simulink model "aerodynamic_model_V1_1_Coupling"  (R2025b)
settings: Solver=ode4  StartTime=0.0  StopTime=8  FixedStep=Ts  RelTol=1e-3
InitFcn:
  | % Run initial_main.m first to load Ad,As,Tq_prop,Tq_mass,...
values from neighbouring files (symbols this model uses):
  alpha_du0_v_tail_L = trim_aero_ic.v_tail_L.alpha_du0    [initial_main_V1_1.m]
  alpha_du0_v_tail_R = trim_aero_ic.v_tail_R.alpha_du0    [initial_main_V1_1.m]
  alpha_du0_wing_L = trim_aero_ic.wing_L.alpha_du0    [initial_main_V1_1.m]
  alpha_du0_wing_R = trim_aero_ic.wing_R.alpha_du0    [initial_main_V1_1.m]
  As = sys_sd.A    [initial_main_V1_1.m]
  BladePitch_deg = 34    [initial_main_V1_1.m]
  Bs = sys_sd.B    [initial_main_V1_1.m]
  Cs = sys_sd.C    [initial_main_V1_1.m]
  ctrl_delta_lim_deg = strips.delta_lim_deg    [initial_main_V1_1.m]
  ctrl_map_aileron_L = aero.wing_L.map_aileron(:)    [initial_main_V1_1.m]
  ctrl_map_aileron_R = aero.wing_R.map_aileron(:)    [initial_main_V1_1.m]
  ctrl_map_tail_L = aero.v_tail_L.map_tail(:)    [initial_main_V1_1.m]
  ctrl_map_tail_R = aero.v_tail_R.map_tail(:)    [initial_main_V1_1.m]
  Ds = sys_sd.D    [initial_main_V1_1.m]
  I_cg_b = R_sb * I_cg_m * R_sb.'    [aeroelastic.m]    (also in initial_main_V1_1.m = grav.I_cg_b)
  I_cg_b_inv = R_sb * I_cg_m_inv * R_sb.'    [aeroelastic.m]    (also in initial_main_V1_1.m = grav.I_cg_b_inv)
  m_total_kg = grav.m_total_kg    [initial_main_V1_1.m]
  n_modes = size(Phi, 2)    [aeroelastic.m]    (also in initial_main_V1_1.m = n_rigid + n_elastic)
  ones_1_tail = ones(1, size(r_cg2ac_b_v_tail_L, 2))    [initial_main_V1_1.m]
  ones_1_wing = ones(1, size(r_cg2ac_b_wing_L, 2))    [initial_main_V1_1.m]
  polar_alpha_deg = polar.alpha_deg(:).'    [initial_main_V1_1.m]
  polar_CD = polar.CD(:).'    [initial_main_V1_1.m]
  polar_CDp = polar.CDp(:).'    [initial_main_V1_1.m]
  polar_CL = polar.CL(:).'    [initial_main_V1_1.m]
  polar_CM = polar.CM(:).'    [initial_main_V1_1.m]
  r_cg2ac_b_v_tail_L = R_sb * aero.v_tail_L.r_ac_s    [initial_main_V1_1.m]
  r_cg2ac_b_v_tail_R = R_sb * aero.v_tail_R.r_ac_s    [initial_main_V1_1.m]
  r_cg2ac_b_wing_L = R_sb * aero.wing_L.r_ac_s    [initial_main_V1_1.m]
  r_cg2ac_b_wing_R = R_sb * aero.wing_R.r_ac_s    [initial_main_V1_1.m]
  r_cg2kink_b = eng.r_cg2kink_b    [initial_main_V1_1.m]
  r_cg2node_b = aeroelastic.node_arms(nodes, 'R_sb', R_sb).r_cg2node_b    [initial_main_V1_1.m]
  T_aero2W = aeroelastic.wing_aileron_to_W(strips).T    [initial_main_V1_1.m]
  T_prop2W = load_maps.T_prop2W    [initial_main_V1_1.m]
  Tq_mass = load_maps.Tq_mass    [initial_main_V1_1.m]
  trim_Attitude_rad0 = trim_default.Attitude_rad0    [initial_main_V1_1.m]
  trim_Omega_b0 = trim_default.Omega_b0    [initial_main_V1_1.m]
  trim_Position0 = trim_default.Position0    [initial_main_V1_1.m]
  trim_Velocity_b0 = trim_default.Velocity_b0    [initial_main_V1_1.m]
  Ts = 0.001    [initial_main_V1_1.m]
  U = 50    [initial_main_V1_1.m]
  v_tail_cant_rad = deg2rad(v_tail_cant_deg)    [initial_main_V1_1.m]
  W_mass_g = grav.W_mass    [initial_main_V1_1.m]
  x0_structure = trim_default.x0_structure    [initial_main_V1_1.m]
  x0_wagner_v_tail_L = trim_aero_ic.v_tail_L.x0_wagner    [initial_main_V1_1.m]
  x0_wagner_v_tail_R = trim_aero_ic.v_tail_R.x0_wagner    [initial_main_V1_1.m]
  x0_wagner_wing_L = trim_aero_ic.wing_L.x0_wagner    [initial_main_V1_1.m]
  x0_wagner_wing_R = trim_aero_ic.wing_R.x0_wagner    [initial_main_V1_1.m]
undefined symbols (not defined in the file or in its folder): Ad_v_tail_L, Ad_v_tail_R, Ad_wing_L, Ad_wing_R, Bd_v_tail_L, Bd_v_tail_R, Bd_wing_L, Bd_wing_R, c_over_2U_v_tail_L, c_over_2U_v_tail_R, c_over_2U_wing_L, c_over_2U_wing_R, Cd_v_tail_L, Cd_v_tail_R, Cd_wing_L, Cd_wing_R, Dd_v_tail_L, Dd_v_tail_R, Dd_wing_L, Dd_wing_R, G_du_v_tail_L, G_du_v_tail_R, G_du_wing_L, G_du_wing_R, polar_aileron_alpha_deg, polar_aileron_dCD, polar_aileron_dCL, polar_aileron_dCM, polar_aileron_delta_deg, polar_ruddervator_alpha_deg, polar_ruddervator_dCD, polar_ruddervator_dCL, polar_ruddervator_dCM, polar_ruddervator_delta_deg, qS_strip_v_tail_L, qS_strip_v_tail_R, qS_strip_wing_L, qS_strip_wing_R, qSc_strip_v_tail_L, qSc_strip_v_tail_R, qSc_strip_wing_L, qSc_strip_wing_R, T_m2b_v_tail_L, T_m2b_v_tail_R, T_m2b_wing_L, T_m2b_wing_R, T_m2h_v_tail_L, T_m2h_v_tail_R, T_m2h_wing_L, T_m2h_wing_R, Tq_CM_v_tail_L, Tq_CM_v_tail_R, Tq_CM_wing_L, Tq_CM_wing_R, Tq_D_v_tail_L, Tq_D_v_tail_R, Tq_D_wing_L, Tq_D_wing_R, Tq_v_tail_L, Tq_v_tail_R ... (+2)
libraries: Prop_gryo x9, matrix_library x2
(part 1 of 2)
settings Model: Creator=someone  LastModifiedBy=someone
settings DataIOCC: ExternalInput=trim_input_dataset  LoadExternalInput=on

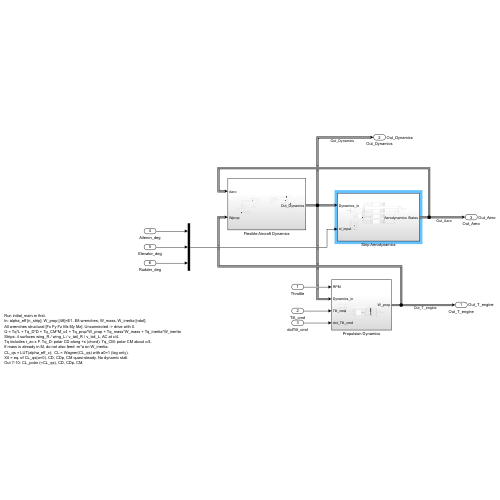
[thumbnail: Simulink's stored preview of the top-level diagram]
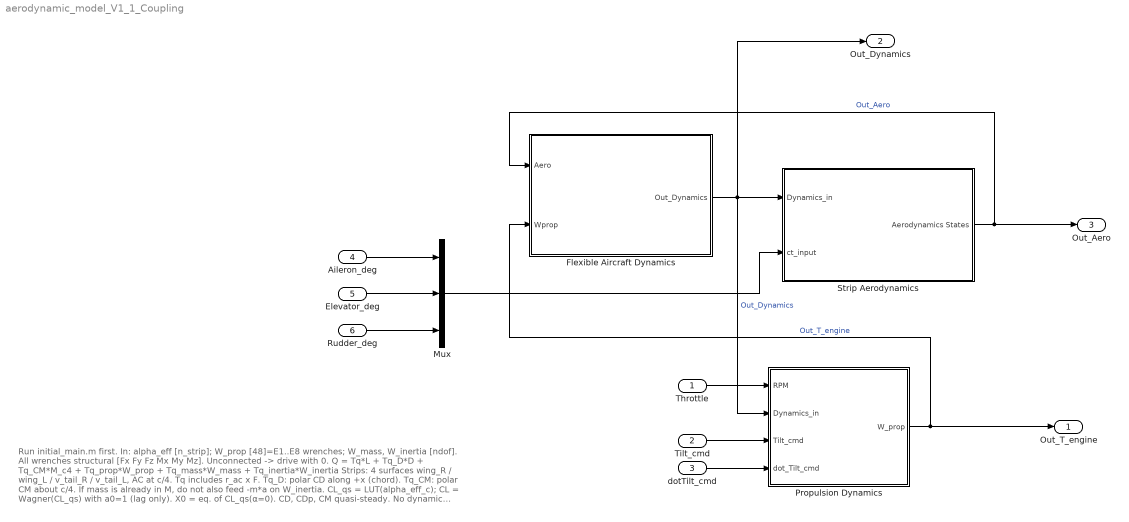
== system aerodynamic_model_V1_1_Coupling ==
  note: Run initial_main.m first.
      | In: alpha_eff [n_strip]; W_prop [48]=E1..E8 wrenches; W_mass, W_inertia [ndof].
      | All wrenches structural [Fx Fy Fz Mx My Mz]. Unconnected -> drive with 0.
      | Q = Tq*L + Tq_D*D + Tq_CM*M_c4 + Tq_prop*W_prop + Tq_mass*W_mass + Tq_inertia*W_inertia
      | Strips: 4 surfaces wing_R / wing_L / v_tail_R / v_tail_L, AC at c/4.
      | Tq includes r_ac x F. Tq_D: polar CD along +x (chord). Tq_CM: polar CM about c/4.
      | If mass is already in M, do not also feed -m*a on W_inertia.
      | CL_qs = LUT(alpha_eff_c);  CL = Wagner(CL_qs) with a0=1 (lag only).
      | X0 = eq. of CL_qs(α=0). CD, CDp, CM quasi-steady. No dynamic stall.
      | Out 7-10: CL_polar (=CL_qs), CD, CDp, CM.
  Throttle : Inport  PortDimensions=8
  Tilt_cmd : Inport  Port=2  PortDimensions=8
  dotTilt_cmd : Inport  Port=3  PortDimensions=8
  Aileron_deg : Inport  Port=4
  Elevator_deg : Inport  Port=5
  Rudder_deg : Inport  Port=6
  Flexible Aircraft Dynamics : Subsystem
  Mux : Mux  Inputs=3
  Propulsion Dynamics : Subsystem
  Strip Aerodynamics : Subsystem
  Out_T_engine : Outport  SignalName=Out_T_engine
  Out_Dynamics : Outport  Port=2  SignalName=Out_Dynamics
  Out_Aero : Outport  Port=3  SignalName=Out_Aero
  wires:
  Throttle/1 -> Propulsion Dynamics/1(RPM)
  Tilt_cmd/1 -> Propulsion Dynamics/3(Tilt_cmd)
  dotTilt_cmd/1 -> Propulsion Dynamics/4(dot_Tilt_cmd)
  Flexible Aircraft Dynamics/1(Out_Dynamics) -> Out_Dynamics/1, Strip Aerodynamics/1(Dynamics_in), Propulsion Dynamics/2(Dynamics_in)  "Out_Dynamics"
  Strip Aerodynamics/1(Aerodynamics States) -> Out_Aero/1, Flexible Aircraft Dynamics/1(Aero)  "Out_Aero"
  Propulsion Dynamics/1(W_prop) -> Out_T_engine/1, Flexible Aircraft Dynamics/2(Wprop)  "Out_T_engine"
  Aileron_deg/1 -> Mux/1
  Rudder_deg/1 -> Mux/3
  Mux/1 -> Strip Aerodynamics/2(ct_input)
  Elevator_deg/1 -> Mux/2

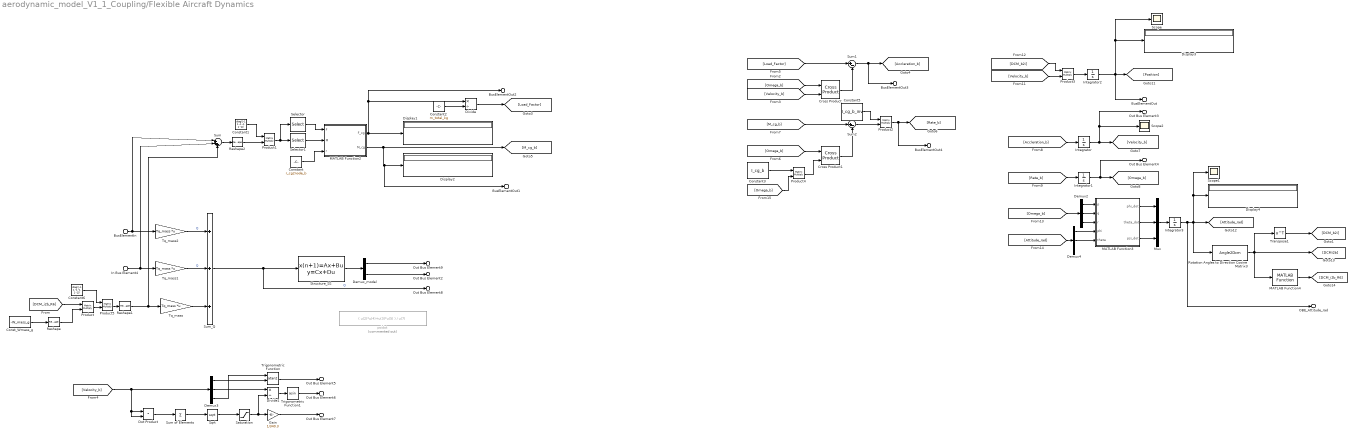
== system aerodynamic_model_V1_1_Coupling/Flexible Aircraft Dynamics ==
  BusElementIn : Inport  PortName=Aero  Element=W_aero_S
  In Bus Element4 : Inport  Port=2  PortName=Wprop  Element=W_m
  Const_Wmass_g : Constant  Value=-W_mass_g
  Constant : Constant  Value=r_cg2node_b
  Constant1 : Constant  Value=diag([-1 1 -1 -1 1 -1])
  Constant2 : Constant  Value=m_total_kg
  Constant3 : Constant  Value=I_cg_b
  Constant5 : Constant  Value=I_cg_b_inv
  Constant6 : Constant  Value=diag([-1 1 -1 -1 1 -1])
  Cross Product : matrix_library/Cross Product
  Cross Product1 : matrix_library/Cross Product
  Demux2 : Demux  Outputs=3
  Demux3 : Demux  Outputs=3
  Demux4 : Demux  Outputs=3
  Demux_modal : Demux  Outputs=[n_modes n_modes]
  Display{1..4} (4 alike) : Display
  Divide : Product  Inputs=*/
  Divide1 : Product  Inputs=*/
  Dot Product : DotProduct  OutDataTypeStr=Inherit: Inherit via internal rule
  Gain : Gain  Gain=1/340.3
  Integrator : Integrator  InitialCondition=trim_Velocity_b0
  Integrator1 : Integrator  InitialCondition=trim_Omega_b0
  Integrator2 : Integrator  InitialCondition=trim_Position0
  Integrator3 : Integrator  InitialCondition=trim_Attitude_rad0
  MATLAB Function2 : MATLAB Function  TreatAsAtomicUnit=on
  MATLAB Function3 : MATLAB Function  TreatAsAtomicUnit=on
  MATLAB Function4 : Prop_gryo/Prop1/MATLAB Function  SystemSampleTime=-1  VariantActivationTime=update diagram  EmptyChoice=off  PassThrough=off  PassThroughVariantControl=(default)  EmptyChoiceVariantControl=(default)  AllowFlexibleInterface=on  Latency=0  AutoFrameSizeCalculation=off
  Mux : Mux  Inputs=3
  Product{,1..5} (6 alike) : Product  Multiplication=Matrix(*)
  Reshape : Reshape  OutputDimensionality=Customize  OutputDimensions=[6 89]
  Reshape1 : Reshape
  Reshape2 : Reshape  OutputDimensionality=Customize  OutputDimensions=[6 89]
  Rotation Angles to Direction Cosine Matrix3 : Angle2Dcm
      settings: AttributesFormatString=Rotation Order: %<rotationOrder>
  Saturation : Saturate  UpperLimit=inf  LowerLimit=1e-6
  Scope : Scope
      settings: ActiveDisplayYMinimum=-1  ActiveDisplayYMaximum=1
  Scope1 : Scope
      settings: ActiveDisplayYMinimum=-1  ActiveDisplayYMaximum=1
  Scope2 : Scope
      settings: ActiveDisplayYMinimum=-1  ActiveDisplayYMaximum=1  DataLoggingVariableName=ScopeData2
  Selector : Selector  NumberOfDimensions=2  InputPortWidth=3  IndexOptions=Index vector (dialog),Index vector (dialog)  Indices=[1:3],[1:89]  OutputSizes=1,1
  Selector1 : Selector  NumberOfDimensions=2  InputPortWidth=3  IndexOptions=Index vector (dialog),Index vector (dialog)  Indices=[4:6],[1:89]  OutputSizes=1,1
  Sqrt : Sqrt
  Structure_SS : DiscreteStateSpace  A=As  B=Bs  C=Cs  D=Ds  InitialCondition=x0_structure  SampleTime=Ts
  Sum : Sum  Inputs=|+++
  Sum of Elements : Sum  Inputs=+
  Sum1 : Sum  Inputs=|+-
  Sum2 : Sum  Inputs=|+-
  Sum_Q : Sum  Inputs=+++
  Tq_mass : Gain  Gain=Tq_mass  Multiplication=Matrix(K*u)
  Tq_mass1 : Gain  Gain=Tq_mass  Multiplication=Matrix(K*u)
  Tq_mass2 : Gain  Gain=Tq_mass  Multiplication=Matrix(K*u)
  Transpose1 : Math  Operator=transpose
  Trigonometric Function : Trigonometry  Operator=atan2
  Trigonometric Function1 : Trigonometry  Operator=asin
  psidot : Fcn  Commented=on  Expr=( u(2)*u(4)+u(3)*u(5) ) / u(7)
  Out Bus Element2 : Outport  PortName=Out_Dynamics  Element=elastic_m_velocity
  Out Bus Element3 : Outport  PortName=Out_Dynamics  Element=Velocity_b
  Out Bus Element4 : Outport  PortName=Out_Dynamics  Element=Omega_b
  Out Bus Element5 : Outport  PortName=Out_Dynamics  Element=Alpha
  Out Bus Element6 : Outport  PortName=Out_Dynamics  Element=Beta
  Out Bus Element7 : Outport  PortName=Out_Dynamics  Element=mach
  Out Bus Element8 : Outport  PortName=Out_Dynamics  Element=Q
  Out Bus Element9 : Outport  PortName=Out_Dynamics  Element=elastic_displacement
  OBE_Attitude_rad : Outport  PortName=Out_Dynamics  Element=Attitude_rad
  BusElementOut : Outport  PortName=Out_Dynamics  Element=Position
  BusElementOut1 : Outport  PortName=Out_Dynamics  Element=M_cg
  BusElementOut2 : Outport  PortName=Out_Dynamics  Element=F_cg
  BusElementOut3 : Outport  PortName=Out_Dynamics  Element=Acc_b
  BusElementOut4 : Outport  PortName=Out_Dynamics  Element=Rate_b
  wires:
  Dot Product/1 -> Sum of Elements/1
  [Velocity_b] -> Demux3/1, Dot Product/2, Dot Product/1
  Demux3/3 -> Trigonometric Function/1
  Sum_Q/1 -> Structure_SS/1, Out Bus Element8/1  "Q"
  In Bus Element4/1 -> Tq_mass1/1, Sum/2
  Demux_modal/2 -> Out Bus Element2/1
  Demux_modal/1 -> Out Bus Element9/1
  Tq_mass/1 -> Sum_Q/3
  Sum of Elements/1 -> Sqrt/1
  Demux3/2 -> Divide1/1
  Structure_SS/1 -> Demux_modal/1
  Divide1/1 -> Trigonometric Function1/1
  Demux3/1 -> Trigonometric Function/2
  Const_Wmass_g/1 -> Reshape/1
  Sqrt/1 -> Saturation/1
  Saturation/1 -> Gain/1, Divide1/2
  Trigonometric Function/1 -> Out Bus Element5/1
  Trigonometric Function1/1 -> Out Bus Element6/1
  Gain/1 -> Out Bus Element7/1
  Tq_mass1/1 -> Sum_Q/2  "Q"
  BusElementIn/1 -> Sum/1, Tq_mass2/1
  Tq_mass2/1 -> Sum_Q/1  "Q"
  [DCM_i2b_R6] -> Product/1
  Reshape/1 -> Product/2
  Product5/1 -> Reshape1/1
  Reshape1/1 -> Tq_mass/1, Sum/3
  Sum/1 -> Reshape2/1
  Reshape2/1 -> Product1/2
  Selector/1 -> MATLAB Function2/1(F)
  Selector1/1 -> MATLAB Function2/2(M)
  Constant/1 -> MATLAB Function2/3(r)
  Constant1/1 -> Product1/1
  Product1/1 -> Selector1/1, Selector/1
  MATLAB Function2/1(F_cg) -> Divide/1, BusElementOut2/1, Display1/1
  MATLAB Function2/2(M_cg) -> BusElementOut1/1, Display2/1, [M_cg_b]
  [Omega_b] -> Cross Product/1
  [Velocity_b] -> Cross Product/2
  [Load_Factor] -> Sum1/1
  Cross Product/1 -> Sum1/2
  Constant2/1 -> Divide/2
  Divide/1 -> [Load_Factor]
  Sum1/1 -> BusElementOut3/1, [Accleration_b]
  [Omega_b] -> Cross Product1/1
  Constant3/1 -> Product4/1
  [M_cg_b] -> Sum2/1
  Cross Product1/1 -> Sum2/2
  [Accleration_b] -> Integrator/1
  [Rate_b] -> Integrator1/1
  Integrator/1 -> Scope2/1, Out Bus Element3/1, [Velocity_b]
  Integrator1/1 -> Out Bus Element4/1, [Omega_b]
  Sum2/1 -> Product2/2
  Constant5/1 -> Product2/1
  Product2/1 -> BusElementOut4/1, [Rate_b]
  [Velocity_b] -> Product3/2
  [DCM_b2i] -> Product3/1
  Product3/1 -> Integrator2/1
  Integrator2/1 -> BusElementOut/1, Display3/1, Scope/1, [Position]
  Integrator3/1 -> Rotation Angles to Direction Cosine Matrix3/1, Scope1/1, Display4/1, [Attitude_rad], OBE_Attitude_rad/1
  [Omega_b] -> Demux2/1
  Demux2/1 -> MATLAB Function3/1(p)
  Demux2/2 -> MATLAB Function3/2(q)
  Demux2/3 -> MATLAB Function3/3(r)
  [Attitude_rad] -> Demux4/1
  Demux4/1 -> MATLAB Function3/4(phi)
  Demux4/2 -> MATLAB Function3/5(theta)
  Mux/1 -> Integrator3/1
  MATLAB Function3/1(phi_dot) -> Mux/1
  MATLAB Function3/2(theta_dot) -> Mux/2
  MATLAB Function3/3(psi_dot) -> Mux/3
  [Omega_b] -> Product4/2
  Product4/1 -> Cross Product1/2
  Rotation Angles to Direction Cosine Matrix3/1 -> Transpose1/1, MATLAB Function4/1, [DCMi2b]
  MATLAB Function4/1 -> [DCM_i2b_R6]
  Transpose1/1 -> [DCM_b2i]
  Constant6/1 -> Product5/1
  Product/1 -> Product5/2

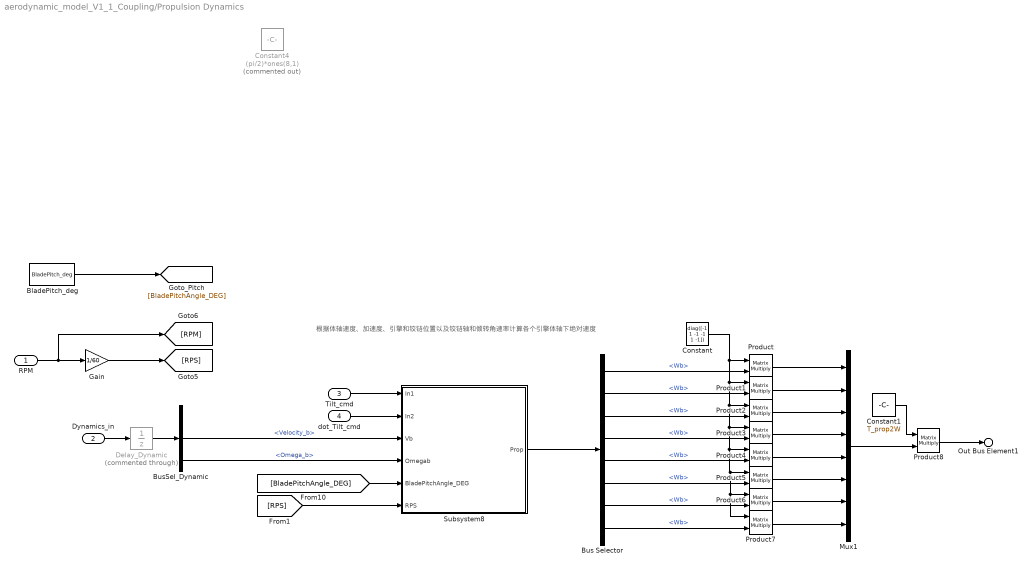
== system aerodynamic_model_V1_1_Coupling/Propulsion Dynamics ==
  note: 根据体轴速度、加速度、引擎和铰链位置以及铰链轴和倾转角速率计算各个引擎体轴下绝对速度
  RPM : Inport  PortDimensions=8
  Dynamics_in : Inport  Port=2
  Tilt_cmd : Inport  Port=3  PortDimensions=8
  dot_Tilt_cmd : Inport  Port=4  PortDimensions=8
  BladePitch_deg : Constant  Value=BladePitch_deg
  Bus Selector : BusSelector  OutputSignals=signal1.Wb,signal2.Wb,signal3.Wb,signal4.Wb,signal5.Wb,signal6.Wb,signal7.Wb,signal8.Wb
  BusSel_Dynamic : BusSelector  OutputSignals=mach,Velocity_b,Omega_b
  Constant : Constant  Value=diag([-1 1 -1 -1 1 -1])
  Constant1 : Constant  Value=T_prop2W
  Constant4 : Constant  Commented=on  Value=(pi/2)*ones(8,1)
  Delay_Dynamic : UnitDelay  Commented=through  SampleTime=Ts  HasFrameUpgradeWarning=on
  Gain : Gain  Gain=1/60
  Mux1 : Mux  Inputs=8
  Product{,1..8} (9 alike) : Product  Multiplication=Matrix(*)
  Subsystem8 : Subsystem
  Out Bus Element1 : Outport  PortName=W_prop  Element=W_m
  wires:
  Dynamics_in/1 -> Delay_Dynamic/1
  Delay_Dynamic/1 -> BusSel_Dynamic/1
  BusSel_Dynamic/2 -> Subsystem8/3(Vb)  "<Velocity_b>"
  BusSel_Dynamic/3 -> Subsystem8/4(Omegab)  "<Omega_b>"
  RPM/1 -> [RPM], Gain/1
  Gain/1 -> [RPS]
  BladePitch_deg/1 -> [BladePitchAngle_DEG]
  Tilt_cmd/1 -> Subsystem8/1(In1)
  dot_Tilt_cmd/1 -> Subsystem8/2(In2)
  [BladePitchAngle_DEG] -> Subsystem8/5(BladePitchAngle_DEG)
  [RPS] -> Subsystem8/6(RPS)
  Subsystem8/1(Prop) -> Bus Selector/1
  Constant/1 -> Product7/1, Product6/1, Product5/1, Product4/1, Product3/1, Product2/1, Product1/1, Product/1
  Bus Selector/8 -> Product7/2  "<Wb>"
  Bus Selector/7 -> Product6/2  "<Wb>"
  Bus Selector/6 -> Product5/2  "<Wb>"
  Bus Selector/5 -> Product4/2  "<Wb>"
  Bus Selector/4 -> Product3/2  "<Wb>"
  Bus Selector/3 -> Product2/2  "<Wb>"
  Bus Selector/2 -> Product1/2  "<Wb>"
  Product/1 -> Mux1/1
  Product1/1 -> Mux1/2
  Product2/1 -> Mux1/3
  Product3/1 -> Mux1/4
  Product4/1 -> Mux1/5
  Product5/1 -> Mux1/6
  Product6/1 -> Mux1/7
  Product7/1 -> Mux1/8
  Mux1/1 -> Product8/2
  Constant1/1 -> Product8/1
  Product8/1 -> Out Bus Element1/1
  Bus Selector/1 -> Product/2  "<Wb>"

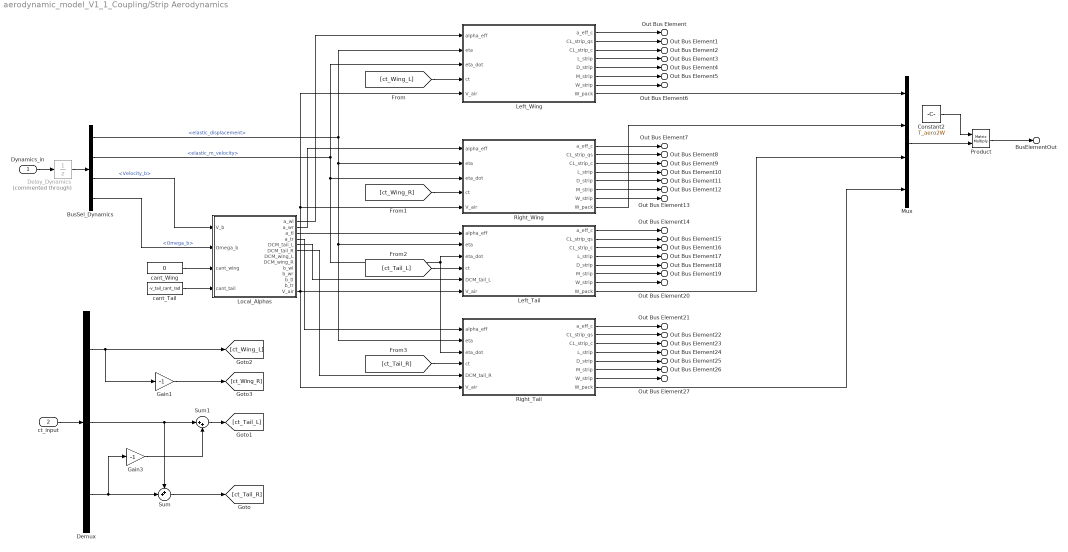
== system aerodynamic_model_V1_1_Coupling/Strip Aerodynamics ==
  Dynamics_in : Inport
  ct_input : Inport  Port=2
  BusSel_Dynamics : BusSelector  OutputSignals=elastic_displacement,elastic_m_velocity,Velocity_b,Omega_b
  Constant2 : Constant  Value=T_aero2W
  Delay_Dynamics : UnitDelay  Commented=through  SampleTime=Ts  HasFrameUpgradeWarning=on
  Demux : Demux  Outputs=3
  Gain1 : Gain  Gain=-1
  Gain3 : Gain  Gain=-1
  Left_Tail : Subsystem
  Left_Wing : Subsystem
  Local_Alphas : Subsystem
  Mux : Mux
  Product : Product  Multiplication=Matrix(*)
  Right_Tail : Subsystem
  Right_Wing : Subsystem
  Sum : Sum  Inputs=++|
  Sum1 : Sum  Inputs=|++
  cant_Tail : Constant  Value=-v_tail_cant_rad
  cant_Wing : Constant  Value=0
  Out Bus Element : Outport  PortName=Aerodynamics States  Element=a_eff_c_LW
  Out Bus Element1 : Outport  PortName=Aerodynamics States  Element=CL_strip_qs_LW
  Out Bus Element2 : Outport  PortName=Aerodynamics States  Element=CL_strip_c_LW
  Out Bus Element3 : Outport  PortName=Aerodynamics States  Element=L_strip_LW
  Out Bus Element4 : Outport  PortName=Aerodynamics States  Element=D_strip_LW
  Out Bus Element5 : Outport  PortName=Aerodynamics States  Element=M_strip_LW
  Out Bus Element6 : Outport  PortName=Aerodynamics States  Element=W_strip_LW
  Out Bus Element7 : Outport  PortName=Aerodynamics States  Element=a_eff_c_RW
  Out Bus Element8 : Outport  PortName=Aerodynamics States  Element=CL_strip_qs_RW
  Out Bus Element9 : Outport  PortName=Aerodynamics States  Element=CL_strip_c_RW
  Out Bus Element10 : Outport  PortName=Aerodynamics States  Element=L_strip_RW
  Out Bus Element11 : Outport  PortName=Aerodynamics States  Element=D_strip_RW
  Out Bus Element12 : Outport  PortName=Aerodynamics States  Element=M_strip_RW
  Out Bus Element13 : Outport  PortName=Aerodynamics States  Element=W_strip_RW
  Out Bus Element14 : Outport  PortName=Aerodynamics States  Element=a_eff_c_LT
  Out Bus Element15 : Outport  PortName=Aerodynamics States  Element=CL_strip_qs_LT
  Out Bus Element16 : Outport  PortName=Aerodynamics States  Element=CL_strip_c_LT
  Out Bus Element17 : Outport  PortName=Aerodynamics States  Element=L_strip_LT
  Out Bus Element18 : Outport  PortName=Aerodynamics States  Element=D_strip_LT
  Out Bus Element19 : Outport  PortName=Aerodynamics States  Element=M_strip_LT
  Out Bus Element20 : Outport  PortName=Aerodynamics States  Element=W_strip_LT
  Out Bus Element21 : Outport  PortName=Aerodynamics States  Element=a_eff_c_RT
  Out Bus Element22 : Outport  PortName=Aerodynamics States  Element=CL_strip_qs_RT
  Out Bus Element23 : Outport  PortName=Aerodynamics States  Element=CL_strip_c_RT
  Out Bus Element24 : Outport  PortName=Aerodynamics States  Element=L_strip_RT
  Out Bus Element25 : Outport  PortName=Aerodynamics States  Element=D_strip_RT
  Out Bus Element26 : Outport  PortName=Aerodynamics States  Element=M_strip_RT
  Out Bus Element27 : Outport  PortName=Aerodynamics States  Element=W_strip_RT
  BusElementOut : Outport  PortName=Aerodynamics States  Element=W_aero_S
  wires:
  Left_Wing/6(M_strip) -> Out Bus Element5/1
  Left_Wing/5(D_strip) -> Out Bus Element4/1
  Left_Wing/4(L_strip) -> Out Bus Element3/1
  Left_Wing/3(CL_strip_c) -> Out Bus Element2/1
  Left_Wing/2(CL_strip_qs) -> Out Bus Element1/1
  Left_Wing/1(a_eff_c) -> Out Bus Element/1
  Left_Wing/7(W_strip) -> Out Bus Element6/1
  Right_Wing/7(W_strip) -> Out Bus Element13/1
  Right_Wing/6(M_strip) -> Out Bus Element12/1
  Right_Wing/5(D_strip) -> Out Bus Element11/1
  Right_Wing/4(L_strip) -> Out Bus Element10/1
  Right_Wing/3(CL_strip_c) -> Out Bus Element9/1
  Right_Wing/2(CL_strip_qs) -> Out Bus Element8/1
  Right_Wing/1(a_eff_c) -> Out Bus Element7/1
  Left_Tail/7(W_strip) -> Out Bus Element20/1
  Left_Tail/6(M_strip) -> Out Bus Element19/1
  Left_Tail/5(D_strip) -> Out Bus Element18/1
  Left_Tail/4(L_strip) -> Out Bus Element17/1
  Left_Tail/3(CL_strip_c) -> Out Bus Element16/1
  Left_Tail/2(CL_strip_qs) -> Out Bus Element15/1
  Left_Tail/1(a_eff_c) -> Out Bus Element14/1
  Right_Tail/7(W_strip) -> Out Bus Element27/1
  Right_Tail/6(M_strip) -> Out Bus Element26/1
  Right_Tail/5(D_strip) -> Out Bus Element25/1
  Right_Tail/4(L_strip) -> Out Bus Element24/1
  Right_Tail/3(CL_strip_c) -> Out Bus Element23/1
  Right_Tail/2(CL_strip_qs) -> Out Bus Element22/1
  Right_Tail/1(a_eff_c) -> Out Bus Element21/1
  Dynamics_in/1 -> Delay_Dynamics/1
  Delay_Dynamics/1 -> BusSel_Dynamics/1
  BusSel_Dynamics/1 -> Left_Wing/2(eta), Right_Tail/2(eta), Left_Tail/2(eta), Right_Wing/2(eta)  "<elastic_displacement>"
  BusSel_Dynamics/2 -> Right_Tail/3(eta_dot), Left_Tail/3(eta_dot), Right_Wing/3(eta_dot), Left_Wing/3(eta_dot)  "<elastic_m_velocity>"
  BusSel_Dynamics/3 -> Local_Alphas/1(V_b)  "<Velocity_b>"
  cant_Wing/1 -> Local_Alphas/3(cant_wing)
  Local_Alphas/1(a_wl) -> Left_Wing/1(alpha_eff)
  Local_Alphas/2(a_wr) -> Right_Wing/1(alpha_eff)
  Local_Alphas/3(a_tl) -> Left_Tail/1(alpha_eff)
  Local_Alphas/4(a_tr) -> Right_Tail/1(alpha_eff)
  ct_input/1 -> Demux/1
  Demux/2 -> Sum/1, Sum1/1
  Sum/1 -> [ct_Tail_R]
  Sum1/1 -> [ct_Tail_L]
  [ct_Wing_L] -> Left_Wing/4(ct)
  [ct_Wing_R] -> Right_Wing/4(ct)
  [ct_Tail_L] -> Left_Tail/4(ct)
  [ct_Tail_R] -> Right_Tail/4(ct)
  Local_Alphas/5(DCM_tail_L) -> Left_Tail/5(DCM_tail_L)
  Local_Alphas/6(DCM_tail_R) -> Right_Tail/5(DCM_tail_R)
  Demux/3 -> Gain3/1, Sum/2
  Gain3/1 -> Sum1/2
  cant_Tail/1 -> Local_Alphas/4(cant_tail)
  Left_Wing/8(W_pack) -> Mux/1
  Mux/1 -> Product/2
  Right_Wing/8(W_pack) -> Mux/2
  Left_Tail/8(W_pack) -> Mux/3
  Right_Tail/8(W_pack) -> Mux/4
  Product/1 -> BusElementOut/1
  Constant2/1 -> Product/1
  BusSel_Dynamics/4 -> Local_Alphas/2(Omega_b)  "<Omega_b>"
  Demux/1 -> Gain1/1, [ct_Wing_L]
  Gain1/1 -> [ct_Wing_R]
  Local_Alphas/13(V_air) -> Right_Wing/5(V_air), Left_Wing/5(V_air), Left_Tail/6(V_air), Right_Tail/6(V_air)

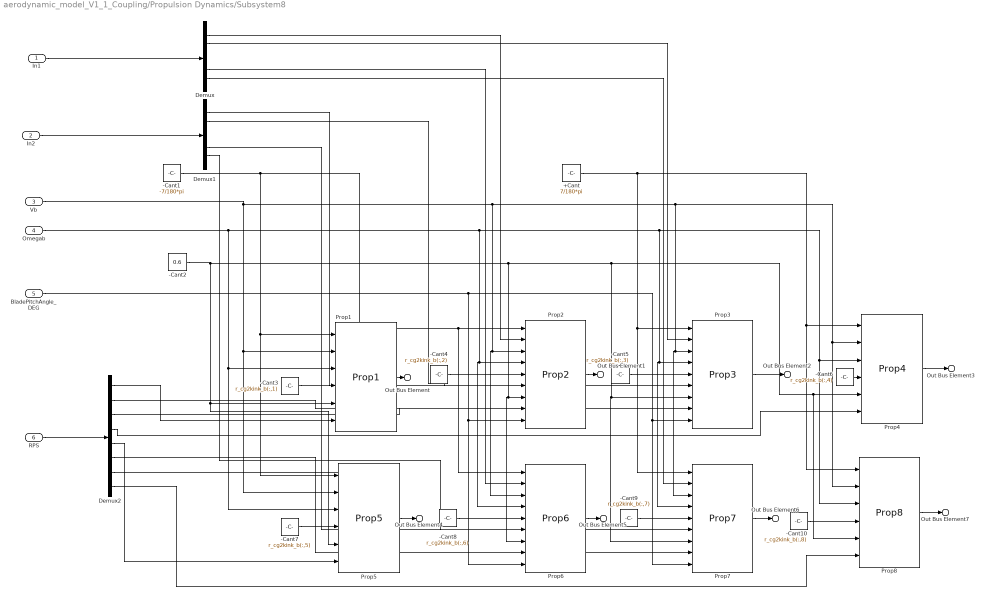
== system aerodynamic_model_V1_1_Coupling/Propulsion Dynamics/Subsystem8 ==
  In1 : Inport
  In2 : Inport  Port=2
  Vb : Inport  Port=3
  Omegab : Inport  Port=4
  BladePitchAngle_DEG : Inport  Port=5
  RPS : Inport  Port=6
  +Cant : Constant  Value=7/180*pi
  -Cant1 : Constant  Value=-7/180*pi
  -Cant10 : Constant  Value=r_cg2kink_b(:,8)
  -Cant2 : Constant  Value=0.6
  -Cant3 : Constant  Value=r_cg2kink_b(:,1)
  -Cant4 : Constant  Value=r_cg2kink_b(:,2)
  -Cant5 : Constant  Value=r_cg2kink_b(:,3)
  -Cant6 : Constant  Value=r_cg2kink_b(:,4)
  -Cant7 : Constant  Value=r_cg2kink_b(:,5)
  -Cant8 : Constant  Value=r_cg2kink_b(:,6)
  -Cant9 : Constant  Value=r_cg2kink_b(:,7)
  Demux : Demux  Outputs=8
  Demux1 : Demux  Outputs=8
  Demux2 : Demux  Outputs=8
  Prop1 : Prop_gryo/Prop1  SystemSampleTime=-1  VariantActivationTime=update diagram  EmptyChoice=off  PassThrough=off  PassThroughVariantControl=(default)  EmptyChoiceVariantControl=(default)  AllowFlexibleInterface=on  Latency=0  AutoFrameSizeCalculation=off
  Prop2 : Prop_gryo/Prop2  SystemSampleTime=-1  VariantActivationTime=update diagram  EmptyChoice=off  PassThrough=off  PassThroughVariantControl=(default)  EmptyChoiceVariantControl=(default)  AllowFlexibleInterface=on  Latency=0  AutoFrameSizeCalculation=off
  Prop3 : Prop_gryo/Prop3  SystemSampleTime=-1  VariantActivationTime=update diagram  EmptyChoice=off  PassThrough=off  PassThroughVariantControl=(default)  EmptyChoiceVariantControl=(default)  AllowFlexibleInterface=on  Latency=0  AutoFrameSizeCalculation=off
  Prop4 : Prop_gryo/Prop4  SystemSampleTime=-1  VariantActivationTime=update diagram  EmptyChoice=off  PassThrough=off  PassThroughVariantControl=(default)  EmptyChoiceVariantControl=(default)  AllowFlexibleInterface=on  Latency=0  AutoFrameSizeCalculation=off
  Prop5 : Prop_gryo/Prop5  SystemSampleTime=-1  VariantActivationTime=update diagram  EmptyChoice=off  PassThrough=off  PassThroughVariantControl=(default)  EmptyChoiceVariantControl=(default)  AllowFlexibleInterface=on  Latency=0  AutoFrameSizeCalculation=off
  Prop6 : Prop_gryo/Prop6  SystemSampleTime=-1  VariantActivationTime=update diagram  EmptyChoice=off  PassThrough=off  PassThroughVariantControl=(default)  EmptyChoiceVariantControl=(default)  AllowFlexibleInterface=on  Latency=0  AutoFrameSizeCalculation=off
  Prop7 : Prop_gryo/Prop7  SystemSampleTime=-1  VariantActivationTime=update diagram  EmptyChoice=off  PassThrough=off  PassThroughVariantControl=(default)  EmptyChoiceVariantControl=(default)  AllowFlexibleInterface=on  Latency=0  AutoFrameSizeCalculation=off
  Prop8 : Prop_gryo/Prop8  SystemSampleTime=-1  VariantActivationTime=update diagram  EmptyChoice=off  PassThrough=off  PassThroughVariantControl=(default)  EmptyChoiceVariantControl=(default)  AllowFlexibleInterface=on  Latency=0  AutoFrameSizeCalculation=off
  Out Bus Element : Outport  PortName=Prop  Element=signal1
  Out Bus Element1 : Outport  PortName=Prop  Element=signal2
  Out Bus Element2 : Outport  PortName=Prop  Element=signal3
  Out Bus Element3 : Outport  PortName=Prop  Element=signal4
  Out Bus Element4 : Outport  PortName=Prop  Element=signal5
  Out Bus Element5 : Outport  PortName=Prop  Element=signal6
  Out Bus Element6 : Outport  PortName=Prop  Element=signal7
  Out Bus Element7 : Outport  PortName=Prop  Element=signal8
  wires:
  In2/1 -> Demux1/1
  -Cant7/1 -> Prop5/4
  Vb/1 -> Prop5/2, Prop1/2, Prop4/2, Prop8/2, Prop7/3, Prop3/3, Prop6/3, Prop2/3
  Demux/7 -> Prop7/2
  Omegab/1 -> Prop5/3, Prop1/3, Prop4/3, Prop8/3, Prop7/4, Prop3/4, Prop6/4, Prop2/4
  Demux1/3 -> Prop3/6
  Demux1/6 -> Prop6/6
  -Cant8/1 -> Prop6/5
  -Cant2/1 -> Prop4/5, Prop8/5, Prop7/7, Prop3/7, Prop6/7, Prop2/7, Prop5/5, Prop1/5
  -Cant1/1 -> Prop5/1, Prop1/1, Prop6/1, Prop2/1
  BladePitchAngle_DEG/1 -> Prop6/9, Prop2/9, Prop3/9, Prop7/9
  -Cant6/1 -> Prop4/4
  Demux1/2 -> Prop2/6
  Demux/6 -> Prop6/2
  -Cant5/1 -> Prop3/5
  -Cant4/1 -> Prop2/5
  +Cant/1 -> Prop4/1, Prop8/1, Prop3/1, Prop7/1
  -Cant3/1 -> Prop1/4
  Demux/2 -> Prop2/2
  -Cant10/1 -> Prop8/4
  Demux1/7 -> Prop7/6
  -Cant9/1 -> Prop7/5
  Demux/3 -> Prop3/2
  In1/1 -> Demux/1
  Prop1/1 -> Out Bus Element/1
  Prop2/1 -> Out Bus Element1/1
  RPS/1 -> Demux2/1
  Demux2/1 -> Prop1/6
  Demux2/2 -> Prop2/8
  Demux2/3 -> Prop3/8
  Demux2/4 -> Prop4/6
  Demux2/5 -> Prop5/6
  Demux2/6 -> Prop6/8
  Demux2/7 -> Prop7/8
  Demux2/8 -> Prop8/6
  Prop3/1 -> Out Bus Element2/1
  Prop4/1 -> Out Bus Element3/1
  Prop5/1 -> Out Bus Element4/1
  Prop6/1 -> Out Bus Element5/1
  Prop8/1 -> Out Bus Element7/1
  Prop7/1 -> Out Bus Element6/1

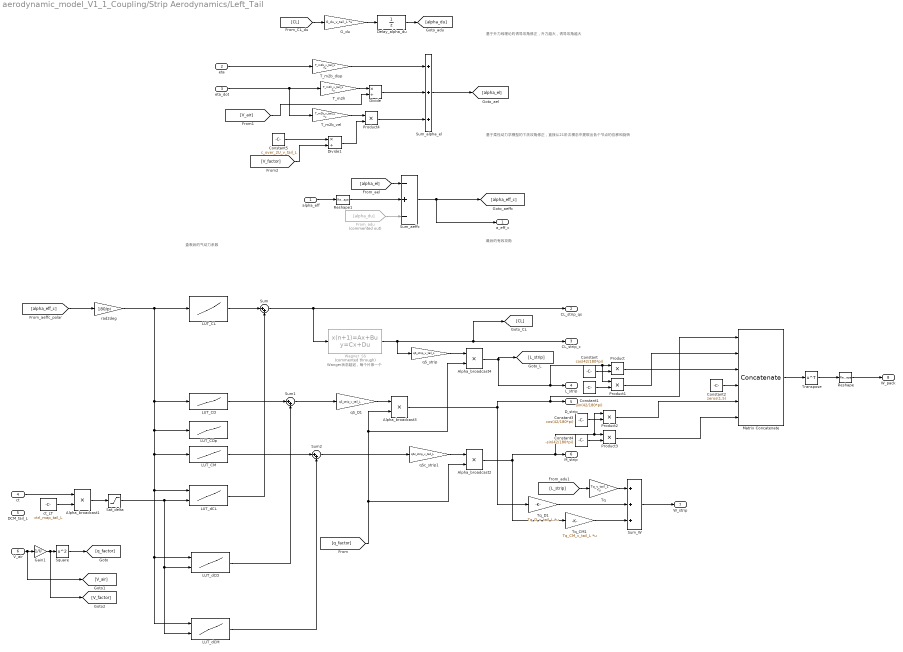
== system aerodynamic_model_V1_1_Coupling/Strip Aerodynamics/Left_Tail ==
  note: 基于升力线理论的诱导攻角修正，升力越大，诱导攻角越大
  note: 基于柔性动力学模型的下洗攻角修正，直接从21阶次模态中提取出各个节点的位移和旋转
  note: 最后的有效攻角
  note: 查表后的气动力系数
  note: Wanger状态延迟，每个片条一个
  alpha_eff : Inport
  eta : Inport  Port=2
  eta_dot : Inport  Port=3
  ct : Inport  Port=4
  DCM_tail_L : Inport  Port=5
  V_air : Inport  Port=6
  Alpha_broadcast{1..4} (4 alike) : Product  Inputs=**
  Constant : Constant  Value=cos(42/180*pi)
  Constant1 : Constant  Value=sin(42/180*pi)
  Constant2 : Constant  Value=zeros(1,5)
  Constant3 : Constant  Value=cos(42/180*pi)
  Constant4 : Constant  Value=-sin(42/180*pi)
  Constant5 : Constant  Value=c_over_2U_v_tail_L
  Delay_alpha_du : UnitDelay  InitialCondition=alpha_du0_v_tail_L  SampleTime=Ts  HasFrameUpgradeWarning=on
  Divide : Product  Inputs=*/
  Divide1 : Product  Inputs=*/
  From_adu : From  Commented=on  GotoTag=alpha_du
  G_du : Gain  Gain=G_du_v_tail_L  Multiplication=Matrix(K*u)
  Gain1 : Gain  Gain=1/U
  LUT_CD : Lookup_n-D  NumberOfTableDimensions=1  BreakpointsForDimension1=polar_alpha_deg  BreakpointsForDimension3=[5, 7]  Table=polar_CD  ExtrapMethod=Clip  InternalRulePriority=Speed  RndMeth=Simplest
  LUT_CDp : Lookup_n-D  NumberOfTableDimensions=1  BreakpointsForDimension1=polar_alpha_deg  BreakpointsForDimension3=[5, 7]  Table=polar_CDp  ExtrapMethod=Clip  InternalRulePriority=Speed  RndMeth=Simplest
  LUT_CL : Lookup_n-D  NumberOfTableDimensions=1  BreakpointsForDimension1=polar_alpha_deg  BreakpointsForDimension3=[5, 7]  Table=polar_CL  ExtrapMethod=Clip  InternalRulePriority=Speed  RndMeth=Simplest
  LUT_CM : Lookup_n-D  NumberOfTableDimensions=1  BreakpointsForDimension1=polar_alpha_deg  BreakpointsForDimension3=[5, 7]  Table=polar_CM  ExtrapMethod=Clip  InternalRulePriority=Speed  RndMeth=Simplest
  LUT_dCD : Lookup_n-D  BreakpointsForDimension1=polar_ruddervator_alpha_deg  BreakpointsForDimension2=polar_ruddervator_delta_deg  BreakpointsForDimension3=[5, 7]  Table=polar_ruddervator_dCD  ExtrapMethod=Clip  InternalRulePriority=Speed  RndMeth=Simplest
      settings: InputPortMap=u0,u1
  LUT_dCL : Lookup_n-D  BreakpointsForDimension1=polar_ruddervator_alpha_deg  BreakpointsForDimension2=polar_ruddervator_delta_deg  BreakpointsForDimension3=[5, 7]  Table=polar_ruddervator_dCL  ExtrapMethod=Clip  InternalRulePriority=Speed  RndMeth=Simplest
      settings: InputPortMap=u0,u1
  LUT_dCM : Lookup_n-D  BreakpointsForDimension1=polar_ruddervator_alpha_deg  BreakpointsForDimension2=polar_ruddervator_delta_deg  BreakpointsForDimension3=[5, 7]  Table=polar_ruddervator_dCM  ExtrapMethod=Clip  InternalRulePriority=Speed  RndMeth=Simplest
      settings: InputPortMap=u0,u1
  Matrix Concatenate : Concatenate  NumInputs=6  Mode=Multidimensional array  ConcatenateDimension=2
  Product{,1..4} (5 alike) : Product
  Reshape : Reshape
  Reshape1 : Reshape
  Sat_delta : Saturate  UpperLimit=ctrl_delta_lim_deg  LowerLimit=-ctrl_delta_lim_deg
  Square : Math  Operator=square
  Sum : Sum  Inputs=|++
  Sum1 : Sum  Inputs=|++
  Sum2 : Sum  Inputs=|++
  Sum_W : Sum  Inputs=+++
  Sum_aeffc : Sum  Inputs=-+-
  Sum_alpha_el : Sum  Inputs=+++
  T_m2b_disp : Gain  Gain=T_m2b_v_tail_L  Multiplication=Matrix(K*u)
  T_m2b_vel : Gain  Gain=T_m2b_v_tail_L  Multiplication=Matrix(K*u)
  T_m2h : Gain  Gain=T_m2h_v_tail_L  Multiplication=Matrix(K*u)
  Tq : Gain  Gain=Tq_v_tail_L  Multiplication=Matrix(K*u)
  Tq_CM1 : Gain  Gain=Tq_CM_v_tail_L  Multiplication=Matrix(K*u)
  Tq_D1 : Gain  Gain=Tq_D_v_tail_L  Multiplication=Matrix(K*u)
  Transpose : Math  Operator=transpose
  Wagner_SS : DiscreteStateSpace  Commented=through  A=Ad_v_tail_L  B=Bd_v_tail_L  C=Cd_v_tail_L  D=Dd_v_tail_L  InitialCondition=x0_wagner_v_tail_L  SampleTime=Ts
  ct_LT : Constant  Value=ctrl_map_tail_L
  qS_D1 : Gain  Gain=qS_strip_v_tail_L
  qS_strip : Gain  Gain=qS_strip_v_tail_L
  qSc_strip1 : Gain  Gain=qSc_strip_v_tail_L
  rad2deg : Gain  Gain=180/pi
  a_eff_c : Outport
  CL_strip_qs : Outport  Port=2
  CL_strip_c : Outport  Port=3
  L_strip : Outport  Port=4
  D_strip : Outport  Port=5
  M_strip : Outport  Port=6
  W_strip : Outport  Port=7
  W_pack : Outport  Port=8
  wires:
  rad2deg/1 -> LUT_CD/1, LUT_CDp/1, LUT_dCL/1, LUT_dCM/1, LUT_dCD/1, LUT_CM/1, LUT_CL/1
  Wagner_SS/1 -> CL_strip_c/1, [CL], qS_strip/1
  eta/1 -> T_m2b_disp/1
  Delay_alpha_du/1 -> [alpha_du]
  Sum/1 -> CL_strip_qs/1, Wagner_SS/1
  T_m2b_vel/1 -> Product4/1
  Divide/1 -> Sum_alpha_el/2
  T_m2b_disp/1 -> Sum_alpha_el/1
  G_du/1 -> Delay_alpha_du/1
  Product4/1 -> Sum_alpha_el/3
  Sum_alpha_el/1 -> [alpha_el]
  Sum_aeffc/1 -> a_eff_c/1, [alpha_eff_c]
  [alpha_eff_c] -> rad2deg/1
  T_m2h/1 -> Divide/1
  eta_dot/1 -> T_m2b_vel/1, T_m2h/1
  Sum1/1 -> qS_D1/1
  Sum2/1 -> qSc_strip1/1
  [CL] -> G_du/1
  [alpha_el] -> Sum_aeffc/1
  From_adu/1 -> Sum_aeffc/3
  [L_strip] -> Tq/1
  Tq/1 -> Sum_W/1
  Tq_D1/1 -> Sum_W/2
  Tq_CM1/1 -> Sum_W/3
  Sum_W/1 -> W_strip/1
  alpha_eff/1 -> Reshape1/1
  ct/1 -> Alpha_broadcast1/1
  ct_LT/1 -> Alpha_broadcast1/2
  Alpha_broadcast1/1 -> Sat_delta/1
  LUT_CL/1 -> Sum/1
  LUT_dCL/1 -> Sum/2
  LUT_CD/1 -> Sum1/1
  LUT_dCD/1 -> Sum1/2
  LUT_CM/1 -> Sum2/1
  LUT_dCM/1 -> Sum2/2
  Sat_delta/1 -> LUT_dCL/2, LUT_dCM/2, LUT_dCD/2
  Alpha_broadcast4/1 -> Product1/1, Product/1, L_strip/1, [L_strip]
  Transpose/1 -> Reshape/1
  Reshape/1 -> W_pack/1
  Alpha_broadcast3/1 -> Matrix Concatenate/1, D_strip/1, Tq_D1/1
  Matrix Concatenate/1 -> Transpose/1
  Constant/1 -> Product/2
  Product/1 -> Matrix Concatenate/3
  Constant1/1 -> Product1/2
  Product1/1 -> Matrix Concatenate/2
  Constant2/1 -> Matrix Concatenate/4
  Product2/1 -> Matrix Concatenate/5
  Product3/1 -> Matrix Concatenate/6
  Constant4/1 -> Product3/2
  Constant3/1 -> Product2/2
  Alpha_broadcast2/1 -> Tq_CM1/1, Product2/1, Product3/1, M_strip/1
  Reshape1/1 -> Sum_aeffc/2
  V_air/1 -> [V_air], Gain1/1
  Square/1 -> [q_factor]
  [q_factor] -> Alpha_broadcast3/2, Alpha_broadcast4/2, Alpha_broadcast2/2
  qSc_strip1/1 -> Alpha_broadcast2/1
  qS_D1/1 -> Alpha_broadcast3/1
  qS_strip/1 -> Alpha_broadcast4/1
  [V_factor] -> Divide1/2
  Constant5/1 -> Divide1/1
  Divide1/1 -> Product4/2
  [V_air] -> Divide/2
  Gain1/1 -> [V_factor], Square/1

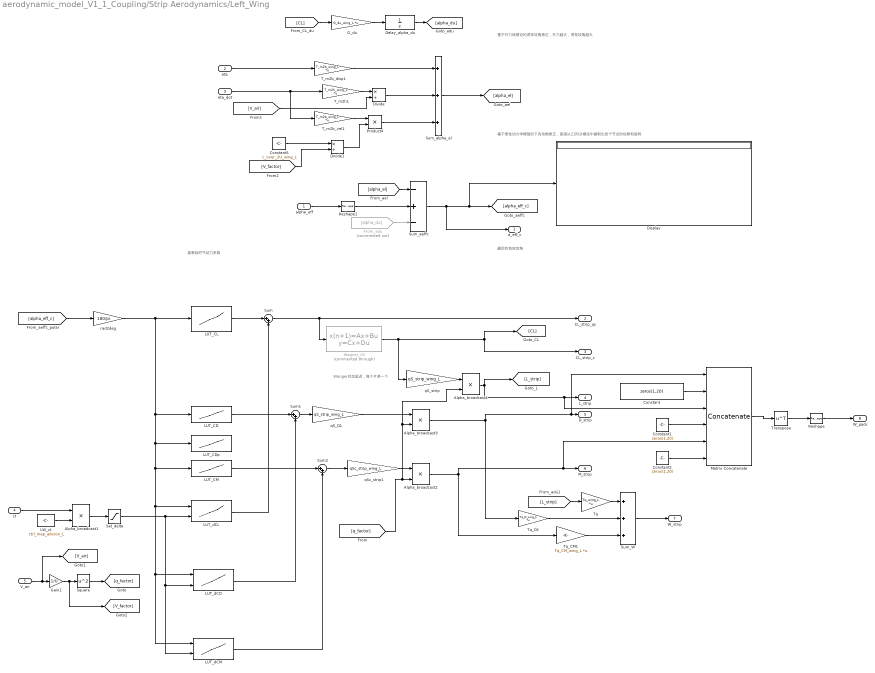
== system aerodynamic_model_V1_1_Coupling/Strip Aerodynamics/Left_Wing ==
  note: 基于升力线理论的诱导攻角修正，升力越大，诱导攻角越大
  note: 基于柔性动力学模型的下洗攻角修正，直接从21阶次模态中提取出各个节点的位移和旋转
  note: 最后的有效攻角
  note: 查表后的气动力系数
  note: Wanger状态延迟，每个片条一个
  alpha_eff : Inport
  eta : Inport  Port=2
  eta_dot : Inport  Port=3
  ct : Inport  Port=4
  V_air : Inport  Port=5
  Alpha_broadcast{1..4} (4 alike) : Product  Inputs=**
  Constant : Constant  Value=zeros(1,20)
  Constant1 : Constant  Value=zeros(1,20)
  Constant2 : Constant  Value=zeros(1,20)
  Constant5 : Constant  Value=c_over_2U_wing_L
  Delay_alpha_du : UnitDelay  InitialCondition=alpha_du0_wing_L  SampleTime=Ts  HasFrameUpgradeWarning=on
  Display : Display
  Divide : Product  Inputs=*/
  Divide1 : Product  Inputs=*/
  From_adu : From  Commented=on  GotoTag=alpha_du
  G_du : Gain  Gain=G_du_wing_L  Multiplication=Matrix(K*u)
  Gain1 : Gain  Gain=1/U
  LUT_CD : Lookup_n-D  NumberOfTableDimensions=1  BreakpointsForDimension1=polar_alpha_deg  BreakpointsForDimension3=[5, 7]  Table=polar_CD  ExtrapMethod=Clip  InternalRulePriority=Speed  RndMeth=Simplest
  LUT_CDp : Lookup_n-D  NumberOfTableDimensions=1  BreakpointsForDimension1=polar_alpha_deg  BreakpointsForDimension3=[5, 7]  Table=polar_CDp  ExtrapMethod=Clip  InternalRulePriority=Speed  RndMeth=Simplest
  LUT_CL : Lookup_n-D  NumberOfTableDimensions=1  BreakpointsForDimension1=polar_alpha_deg  BreakpointsForDimension3=[5, 7]  Table=polar_CL  ExtrapMethod=Clip  InternalRulePriority=Speed  RndMeth=Simplest
  LUT_CM : Lookup_n-D  NumberOfTableDimensions=1  BreakpointsForDimension1=polar_alpha_deg  BreakpointsForDimension3=[5, 7]  Table=polar_CM  ExtrapMethod=Clip  InternalRulePriority=Speed  RndMeth=Simplest
  LUT_dCD : Lookup_n-D  BreakpointsForDimension1=polar_aileron_alpha_deg  BreakpointsForDimension2=polar_aileron_delta_deg  BreakpointsForDimension3=[5, 7]  Table=polar_aileron_dCD  ExtrapMethod=Clip  InternalRulePriority=Speed  RndMeth=Simplest
      settings: InputPortMap=u0,u1
  LUT_dCL : Lookup_n-D  BreakpointsForDimension1=polar_aileron_alpha_deg  BreakpointsForDimension2=polar_aileron_delta_deg  BreakpointsForDimension3=[5, 7]  Table=polar_aileron_dCL  ExtrapMethod=Clip  InternalRulePriority=Speed  RndMeth=Simplest
      settings: InputPortMap=u0,u1
  LUT_dCM : Lookup_n-D  BreakpointsForDimension1=polar_aileron_alpha_deg  BreakpointsForDimension2=polar_aileron_delta_deg  BreakpointsForDimension3=[5, 7]  Table=polar_aileron_dCM  ExtrapMethod=Clip  InternalRulePriority=Speed  RndMeth=Simplest
      settings: InputPortMap=u0,u1
  LW_ct : Constant  Value=ctrl_map_aileron_L
  Matrix Concatenate : Concatenate  NumInputs=6  Mode=Multidimensional array  ConcatenateDimension=2
  Product4 : Product
  Reshape : Reshape
  Reshape1 : Reshape
  Sat_delta : Saturate  UpperLimit=ctrl_delta_lim_deg  LowerLimit=-ctrl_delta_lim_deg
  Square : Math  Operator=square
  Sum : Sum  Inputs=|++
  Sum1 : Sum  Inputs=|++
  Sum2 : Sum  Inputs=|++
  Sum_W : Sum  Inputs=+++
  Sum_aeffc : Sum  Inputs=-+-
  Sum_alpha_el : Sum  Inputs=+++
  T_m2b_disp1 : Gain  Gain=T_m2b_wing_L  Multiplication=Matrix(K*u)
  T_m2b_vel1 : Gain  Gain=T_m2b_wing_L  Multiplication=Matrix(K*u)
  T_m2h1 : Gain  Gain=T_m2h_wing_L  Multiplication=Matrix(K*u)
  Tq : Gain  Gain=Tq_wing_L  Multiplication=Matrix(K*u)
  Tq_CM1 : Gain  Gain=Tq_CM_wing_L  Multiplication=Matrix(K*u)
  Tq_D1 : Gain  Gain=Tq_D_wing_L  Multiplication=Matrix(K*u)
  Transpose : Math  Operator=transpose
  Wagner_SS : DiscreteStateSpace  Commented=through  A=Ad_wing_L  B=Bd_wing_L  C=Cd_wing_L  D=Dd_wing_L  InitialCondition=x0_wagner_wing_L  SampleTime=Ts
  qS_D1 : Gain  Gain=qS_strip_wing_L
  qS_strip : Gain  Gain=qS_strip_wing_L
  qSc_strip1 : Gain  Gain=qSc_strip_wing_L
  rad2deg : Gain  Gain=180/pi
  a_eff_c : Outport
  CL_strip_qs : Outport  Port=2
  CL_strip_c : Outport  Port=3
  L_strip : Outport  Port=4
  D_strip : Outport  Port=5
  M_strip : Outport  Port=6
  W_strip : Outport  Port=7
  W_pack : Outport  Port=8
  wires:
  rad2deg/1 -> LUT_CD/1, LUT_CDp/1, LUT_dCM/1, LUT_dCD/1, LUT_dCL/1, LUT_CM/1, LUT_CL/1
  Wagner_SS/1 -> qS_strip/1, CL_strip_c/1, [CL]
  Delay_alpha_du/1 -> [alpha_du]
  Sum/1 -> CL_strip_qs/1, Wagner_SS/1
  G_du/1 -> Delay_alpha_du/1
  Sum_alpha_el/1 -> [alpha_el]
  Sum_aeffc/1 -> a_eff_c/1, Display/1, [alpha_eff_c]
  [alpha_eff_c] -> rad2deg/1
  Sum1/1 -> qS_D1/1
  Sum2/1 -> qSc_strip1/1
  [CL] -> G_du/1
  [alpha_el] -> Sum_aeffc/1
  From_adu/1 -> Sum_aeffc/3
  Alpha_broadcast2/1 -> Tq_CM1/1, Matrix Concatenate/5, M_strip/1
  [L_strip] -> Tq/1
  Tq/1 -> Sum_W/1
  Tq_D1/1 -> Sum_W/2
  Tq_CM1/1 -> Sum_W/3
  Sum_W/1 -> W_strip/1
  alpha_eff/1 -> Reshape1/1
  ct/1 -> Alpha_broadcast1/1
  LW_ct/1 -> Alpha_broadcast1/2
  Alpha_broadcast1/1 -> Sat_delta/1
  LUT_CL/1 -> Sum/1
  LUT_dCL/1 -> Sum/2
  LUT_CD/1 -> Sum1/1
  LUT_dCD/1 -> Sum1/2
  LUT_CM/1 -> Sum2/1
  LUT_dCM/1 -> Sum2/2
  Sat_delta/1 -> LUT_dCM/2, LUT_dCD/2, LUT_dCL/2
  Alpha_broadcast4/1 -> Matrix Concatenate/3, L_strip/1, [L_strip]
  Alpha_broadcast3/1 -> Tq_D1/1, Matrix Concatenate/1, D_strip/1
  Matrix Concatenate/1 -> Transpose/1
  Transpose/1 -> Reshape/1
  Reshape/1 -> W_pack/1
  Constant/1 -> Matrix Concatenate/2
  Constant1/1 -> Matrix Concatenate/4
  Constant2/1 -> Matrix Concatenate/6
  Reshape1/1 -> Sum_aeffc/2
  V_air/1 -> [V_air], Gain1/1
  Gain1/1 -> [V_factor], Square/1
  Square/1 -> [q_factor]
  qSc_strip1/1 -> Alpha_broadcast2/1
  [q_factor] -> Alpha_broadcast4/2, Alpha_broadcast3/2, Alpha_broadcast2/2
  qS_D1/1 -> Alpha_broadcast3/1
  qS_strip/1 -> Alpha_broadcast4/1
  T_m2b_disp1/1 -> Sum_alpha_el/1
  Product4/1 -> Sum_alpha_el/3
  [V_factor] -> Divide1/2
  Divide/1 -> Sum_alpha_el/2
  Constant5/1 -> Divide1/1
  T_m2h1/1 -> Divide/1
  eta/1 -> T_m2b_disp1/1
  eta_dot/1 -> T_m2b_vel1/1, T_m2h1/1
  Divide1/1 -> Product4/2
  T_m2b_vel1/1 -> Product4/1
  [V_air] -> Divide/2

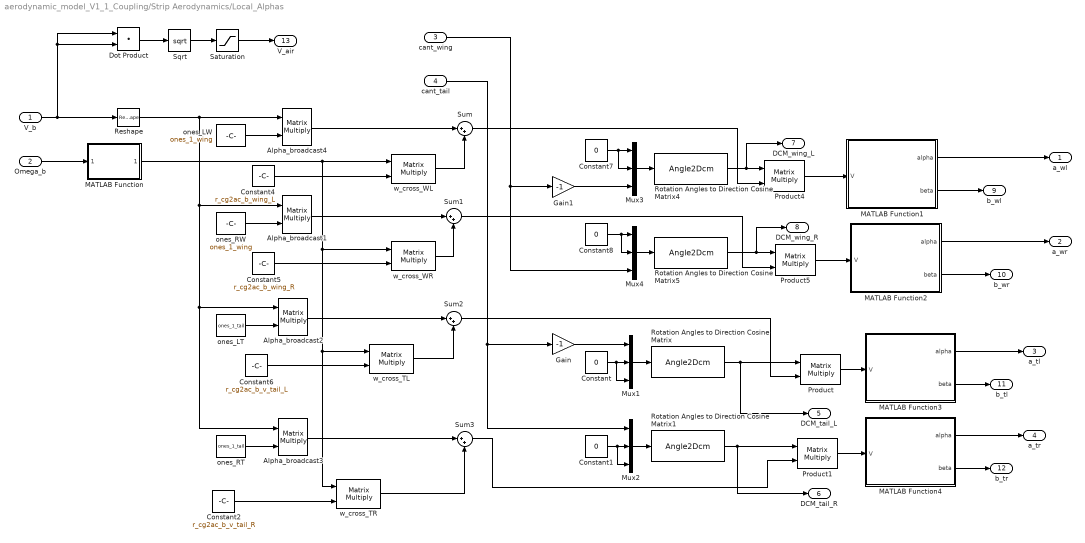
== system aerodynamic_model_V1_1_Coupling/Strip Aerodynamics/Local_Alphas ==
  V_b : Inport  PortDimensions=3
  Omega_b : Inport  Port=2
  cant_wing : Inport  Port=3  PortDimensions=1
  cant_tail : Inport  Port=4
  Alpha_broadcast{1..4} (4 alike) : Product  Multiplication=Matrix(*)
  Constant{,1,7..8} (4 alike) : Constant  Value=0
  Constant2 : Constant  Value=r_cg2ac_b_v_tail_R  VectorParams1D=off
  Constant4 : Constant  Value=r_cg2ac_b_wing_L  VectorParams1D=off
  Constant5 : Constant  Value=r_cg2ac_b_wing_R  VectorParams1D=off
  Constant6 : Constant  Value=r_cg2ac_b_v_tail_L  VectorParams1D=off
  Dot Product : DotProduct  OutDataTypeStr=Inherit: Inherit via internal rule
  Gain : Gain  Gain=-1
  Gain1 : Gain  Gain=-1
  MATLAB Function : MATLAB Function  TreatAsAtomicUnit=on
  MATLAB Function1 : MATLAB Function  TreatAsAtomicUnit=on
  MATLAB Function2 : MATLAB Function  TreatAsAtomicUnit=on
  MATLAB Function3 : MATLAB Function  TreatAsAtomicUnit=on
  MATLAB Function4 : MATLAB Function  TreatAsAtomicUnit=on
  Mux{1..4} (4 alike) : Mux  Inputs=3
  Product{,1,4..5} (4 alike) : Product  Multiplication=Matrix(*)
  Reshape : Reshape  OutputDimensionality=Customize  OutputDimensions=[3 1]
  Rotation Angles to Direction Cosine Matrix{,1,4..5} (4 alike) : Angle2Dcm  rotationOrder=XYZ
      settings: AttributesFormatString=Rotation Order: %<rotationOrder>
  Saturation : Saturate  UpperLimit=inf  LowerLimit=1e-6
  Sqrt : Sqrt
  Sum{,1..3} (4 alike) : Sum  Inputs=|++
  ones_LT : Constant  Value=ones_1_tail  VectorParams1D=off
  ones_LW : Constant  Value=ones_1_wing  VectorParams1D=off
  ones_RT : Constant  Value=ones_1_tail  VectorParams1D=off
  ones_RW : Constant  Value=ones_1_wing  VectorParams1D=off
  w_cross_TL : Product  Multiplication=Matrix(*)
  w_cross_TR : Product  Multiplication=Matrix(*)
  w_cross_WL : Product  Multiplication=Matrix(*)
  w_cross_WR : Product  Multiplication=Matrix(*)
  a_wl : Outport
  a_wr : Outport  Port=2
  a_tl : Outport  Port=3
  a_tr : Outport  Port=4
  DCM_tail_L : Outport  Port=5
  DCM_tail_R : Outport  Port=6
  DCM_wing_L : Outport  Port=7
  DCM_wing_R : Outport  Port=8
  b_wl : Outport  Port=9
  b_wr : Outport  Port=10
  b_tl : Outport  Port=11
  b_tr : Outport  Port=12
  V_air : Outport  Port=13
  wires:
  cant_tail/1 -> Gain/1, Mux2/1
  Gain/1 -> Mux1/1
  Mux1/1 -> Rotation Angles to Direction Cosine Matrix/1
  Mux2/1 -> Rotation Angles to Direction Cosine Matrix1/1
  Constant/1 -> Mux1/3, Mux1/2
  Constant1/1 -> Mux2/3, Mux2/2
  Rotation Angles to Direction Cosine Matrix/1 -> Product/1, DCM_tail_L/1
  Rotation Angles to Direction Cosine Matrix1/1 -> DCM_tail_R/1, Product1/1
  Product/1 -> MATLAB Function3/1(V)
  Product1/1 -> MATLAB Function4/1(V)
  MATLAB Function1/1(alpha) -> a_wl/1
  MATLAB Function1/2(beta) -> b_wl/1
  Sum/1 -> Product4/2
  ones_LW/1 -> Alpha_broadcast4/2
  Alpha_broadcast4/1 -> Sum/1
  ones_RW/1 -> Alpha_broadcast1/2
  Sum1/1 -> Product5/2
  MATLAB Function2/2(beta) -> b_wr/1
  MATLAB Function2/1(alpha) -> a_wr/1
  ones_LT/1 -> Alpha_broadcast2/2
  Alpha_broadcast2/1 -> Sum2/1
  Mux3/1 -> Rotation Angles to Direction Cosine Matrix4/1
  Constant7/1 -> Mux3/2, Mux3/1
  Constant8/1 -> Mux4/2, Mux4/1
  cant_wing/1 -> Mux4/3, Gain1/1
  Gain1/1 -> Mux3/3
  Mux4/1 -> Rotation Angles to Direction Cosine Matrix5/1
  Rotation Angles to Direction Cosine Matrix4/1 -> DCM_wing_L/1, Product4/1
  Product4/1 -> MATLAB Function1/1(V)
  Product5/1 -> MATLAB Function2/1(V)
  Rotation Angles to Direction Cosine Matrix5/1 -> DCM_wing_R/1, Product5/1
  Alpha_broadcast3/1 -> Sum3/1
  ones_RT/1 -> Alpha_broadcast3/2
  Reshape/1 -> Alpha_broadcast4/1, Alpha_broadcast3/1, Alpha_broadcast2/1, Alpha_broadcast1/1
  Sum2/1 -> Product/2
  Sum3/1 -> Product1/2
  MATLAB Function3/1(alpha) -> a_tl/1
  MATLAB Function4/1(alpha) -> a_tr/1
  MATLAB Function3/2(beta) -> b_tl/1
  MATLAB Function4/2(beta) -> b_tr/1
  Alpha_broadcast1/1 -> Sum1/1
  V_b/1 -> Dot Product/2, Dot Product/1, Reshape/1
  Omega_b/1 -> MATLAB Function/1(omega)
  MATLAB Function/1(Omega_skew) -> w_cross_TL/1, w_cross_TR/1, w_cross_WR/1, w_cross_WL/1
  Constant4/1 -> w_cross_WL/2
  w_cross_WL/1 -> Sum/2
  Constant5/1 -> w_cross_WR/2
  w_cross_WR/1 -> Sum1/2
  Constant6/1 -> w_cross_TL/2
  w_cross_TL/1 -> Sum2/2
  Constant2/1 -> w_cross_TR/2
  w_cross_TR/1 -> Sum3/2
  Dot Product/1 -> Sqrt/1
  Sqrt/1 -> Saturation/1
  Saturation/1 -> V_air/1

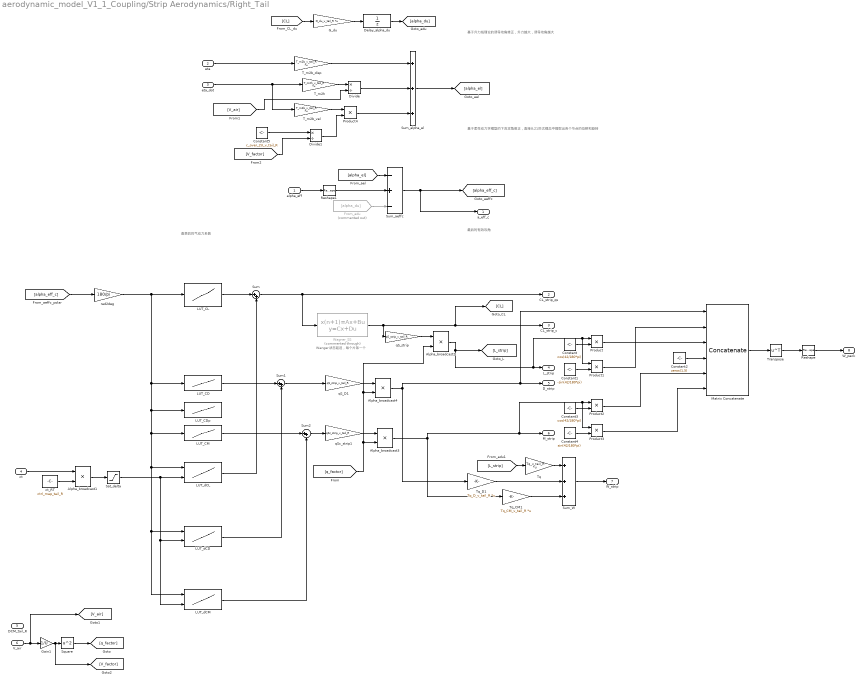
== system aerodynamic_model_V1_1_Coupling/Strip Aerodynamics/Right_Tail ==
  note: Wanger状态延迟，每个片条一个
  note: 查表后的气动力系数
  note: 最后的有效攻角
  note: 基于柔性动力学模型的下洗攻角修正，直接从21阶次模态中提取出各个节点的位移和旋转
  note: 基于升力线理论的诱导攻角修正，升力越大，诱导攻角越大
  alpha_eff : Inport
  eta : Inport  Port=2
  eta_dot : Inport  Port=3
  ct : Inport  Port=4
  DCM_tail_R : Inport  Port=5
  V_air : Inport  Port=6
  Alpha_broadcast{1..4} (4 alike) : Product  Inputs=**
  Constant : Constant  Value=cos(42/180*pi)
  Constant1 : Constant  Value=-sin(42/180*pi)
  Constant2 : Constant  Value=zeros(1,5)
  Constant3 : Constant  Value=cos(42/180*pi)
  Constant4 : Constant  Value=sin(42/180*pi)
  Constant5 : Constant  Value=c_over_2U_v_tail_R
  Delay_alpha_du : UnitDelay  InitialCondition=alpha_du0_v_tail_R  SampleTime=Ts  HasFrameUpgradeWarning=on
  Divide : Product  Inputs=*/
  Divide1 : Product  Inputs=*/
  From_adu : From  Commented=on  GotoTag=alpha_du
  G_du : Gain  Gain=G_du_v_tail_R  Multiplication=Matrix(K*u)
  Gain1 : Gain  Gain=1/U
  LUT_CD : Lookup_n-D  NumberOfTableDimensions=1  BreakpointsForDimension1=polar_alpha_deg  BreakpointsForDimension3=[5, 7]  Table=polar_CD  ExtrapMethod=Clip  InternalRulePriority=Speed  RndMeth=Simplest
  LUT_CDp : Lookup_n-D  NumberOfTableDimensions=1  BreakpointsForDimension1=polar_alpha_deg  BreakpointsForDimension3=[5, 7]  Table=polar_CDp  ExtrapMethod=Clip  InternalRulePriority=Speed  RndMeth=Simplest
  LUT_CL : Lookup_n-D  NumberOfTableDimensions=1  BreakpointsForDimension1=polar_alpha_deg  BreakpointsForDimension3=[5, 7]  Table=polar_CL  ExtrapMethod=Clip  InternalRulePriority=Speed  RndMeth=Simplest
  LUT_CM : Lookup_n-D  NumberOfTableDimensions=1  BreakpointsForDimension1=polar_alpha_deg  BreakpointsForDimension3=[5, 7]  Table=polar_CM  ExtrapMethod=Clip  InternalRulePriority=Speed  RndMeth=Simplest
  LUT_dCD : Lookup_n-D  BreakpointsForDimension1=polar_ruddervator_alpha_deg  BreakpointsForDimension2=polar_ruddervator_delta_deg  BreakpointsForDimension3=[5, 7]  Table=polar_ruddervator_dCD  ExtrapMethod=Clip  InternalRulePriority=Speed  RndMeth=Simplest
      settings: InputPortMap=u0,u1
  LUT_dCL : Lookup_n-D  BreakpointsForDimension1=polar_ruddervator_alpha_deg  BreakpointsForDimension2=polar_ruddervator_delta_deg  BreakpointsForDimension3=[5, 7]  Table=polar_ruddervator_dCL  ExtrapMethod=Clip  InternalRulePriority=Speed  RndMeth=Simplest
      settings: InputPortMap=u0,u1
  LUT_dCM : Lookup_n-D  BreakpointsForDimension1=polar_ruddervator_alpha_deg  BreakpointsForDimension2=polar_ruddervator_delta_deg  BreakpointsForDimension3=[5, 7]  Table=polar_ruddervator_dCM  ExtrapMethod=Clip  InternalRulePriority=Speed  RndMeth=Simplest
      settings: InputPortMap=u0,u1
  Matrix Concatenate : Concatenate  NumInputs=6  Mode=Multidimensional array  ConcatenateDimension=2
  Product{,1..4} (5 alike) : Product
  Reshape : Reshape
  Reshape1 : Reshape
  Sat_delta : Saturate  UpperLimit=ctrl_delta_lim_deg  LowerLimit=-ctrl_delta_lim_deg
  Square : Math  Operator=square
  Sum : Sum  Inputs=|++
  Sum1 : Sum  Inputs=|++
  Sum2 : Sum  Inputs=|++
  Sum_W : Sum  Inputs=+++
  Sum_aeffc : Sum  Inputs=-+-
  Sum_alpha_el : Sum  Inputs=+++
  T_m2b_disp : Gain  Gain=T_m2b_v_tail_R  Multiplication=Matrix(K*u)
  T_m2b_vel : Gain  Gain=T_m2b_v_tail_R  Multiplication=Matrix(K*u)
  T_m2h : Gain  Gain=T_m2h_v_tail_R  Multiplication=Matrix(K*u)
  Tq : Gain  Gain=Tq_v_tail_R  Multiplication=Matrix(K*u)
  Tq_CM1 : Gain  Gain=Tq_CM_v_tail_R  Multiplication=Matrix(K*u)
  Tq_D1 : Gain  Gain=Tq_D_v_tail_R  Multiplication=Matrix(K*u)
  Transpose : Math  Operator=transpose
  Wagner_SS : DiscreteStateSpace  Commented=through  A=Ad_v_tail_R  B=Bd_v_tail_R  C=Cd_v_tail_R  D=Dd_v_tail_R  InitialCondition=x0_wagner_v_tail_R  SampleTime=Ts
  ct_RT : Constant  Value=ctrl_map_tail_R
  qS_D1 : Gain  Gain=qS_strip_v_tail_R
  qS_strip : Gain  Gain=qS_strip_v_tail_R
  qSc_strip1 : Gain  Gain=qSc_strip_v_tail_R
  rad2deg : Gain  Gain=180/pi
  a_eff_c : Outport
  CL_strip_qs : Outport  Port=2
  CL_strip_c : Outport  Port=3
  L_strip : Outport  Port=4
  D_strip : Outport  Port=5
  M_strip : Outport  Port=6
  W_strip : Outport  Port=7
  W_pack : Outport  Port=8
  wires:
  Sat_delta/1 -> LUT_dCL/2, LUT_dCM/2, LUT_dCD/2
  LUT_dCM/1 -> Sum2/2
  LUT_CM/1 -> Sum2/1
  LUT_dCD/1 -> Sum1/2
  LUT_CD/1 -> Sum1/1
  LUT_dCL/1 -> Sum/2
  LUT_CL/1 -> Sum/1
  Alpha_broadcast1/1 -> Sat_delta/1
  ct_RT/1 -> Alpha_broadcast1/2
  ct/1 -> Alpha_broadcast1/1
  alpha_eff/1 -> Reshape1/1
  Sum_W/1 -> W_strip/1
  Tq_CM1/1 -> Sum_W/3
  Tq_D1/1 -> Sum_W/2
  Tq/1 -> Sum_W/1
  [L_strip] -> Tq/1
  From_adu/1 -> Sum_aeffc/3
  [alpha_el] -> Sum_aeffc/1
  [CL] -> G_du/1
  Sum2/1 -> qSc_strip1/1
  Sum1/1 -> qS_D1/1
  [alpha_eff_c] -> rad2deg/1
  Sum_aeffc/1 -> [alpha_eff_c], a_eff_c/1
  Sum_alpha_el/1 -> [alpha_el]
  G_du/1 -> Delay_alpha_du/1
  Sum/1 -> Wagner_SS/1, CL_strip_qs/1
  Delay_alpha_du/1 -> [alpha_du]
  Wagner_SS/1 -> qS_strip/1, [CL], CL_strip_c/1
  rad2deg/1 -> LUT_CL/1, LUT_CM/1, LUT_dCL/1, LUT_dCM/1, LUT_dCD/1, LUT_CDp/1, LUT_CD/1
  Transpose/1 -> Reshape/1
  Reshape/1 -> W_pack/1
  Alpha_broadcast4/1 -> Matrix Concatenate/1, D_strip/1, Tq_D1/1
  Matrix Concatenate/1 -> Transpose/1
  Product/1 -> Matrix Concatenate/3
  Constant1/1 -> Product1/2
  Alpha_broadcast2/1 -> Product1/1, Product/1, L_strip/1, [L_strip]
  Constant/1 -> Product/2
  Product1/1 -> Matrix Concatenate/2
  Constant2/1 -> Matrix Concatenate/4
  Constant4/1 -> Product3/2
  Product3/1 -> Matrix Concatenate/6
  Alpha_broadcast3/1 -> Tq_CM1/1, Product3/1, Product2/1, M_strip/1
  Constant3/1 -> Product2/2
  Product2/1 -> Matrix Concatenate/5
  Reshape1/1 -> Sum_aeffc/2
  Square/1 -> [q_factor]
  V_air/1 -> [V_air], Gain1/1
  [q_factor] -> Alpha_broadcast2/2, Alpha_broadcast4/2, Alpha_broadcast3/2
  qSc_strip1/1 -> Alpha_broadcast3/1
  qS_D1/1 -> Alpha_broadcast4/1
  qS_strip/1 -> Alpha_broadcast2/1
  [V_factor] -> Divide1/2
  Divide1/1 -> Product4/2
  T_m2h/1 -> Divide/1
  T_m2b_vel/1 -> Product4/1
  eta_dot/1 -> T_m2b_vel/1, T_m2h/1
  eta/1 -> T_m2b_disp/1
  Constant5/1 -> Divide1/1
  T_m2b_disp/1 -> Sum_alpha_el/1
  Divide/1 -> Sum_alpha_el/2
  Product4/1 -> Sum_alpha_el/3
  [V_air] -> Divide/2
  Gain1/1 -> [V_factor], Square/1
